simulink model "air_quad"  (R2022b)
settings: Solver=FixedStepDiscrete  StartTime=0.0  StopTime=20  FixedStep=0.01  RelTol=1e-3
model workspace (MAT data in the model file):
  air_quad_config.schema_version = '0.3'
  air_quad_config.plane_model_id = 'quad_sim_b_workbook_b40_v1'
  air_quad_config.power_model_id = 'bench_workbook_fit_v1'
  air_quad_config.power_source = 'bench_synth'
  air_quad_config.mass_kg = 9.581
  air_quad_config.gravity_mps2 = 9.81
  air_quad_config.arm_m = 1
  air_quad_config.rotor_radius_m = 0.508
  air_quad_config.rotor_angle_rad = [0.785398163397; 2.35619449019; 3.92699081699; 5.49778714378]
  air_quad_config.rotor_direction = [1; -1; 1; -1]
  air_quad_config.inertia_kgm2 = [1.3866475  0  0; 0  1.3866475  0; 0  0  2.8184016]
  air_quad_config.pwm_min_us = 1000
  air_quad_config.pwm_max_us = 2000
  air_quad_config.motor_tau_s = 0.08
  air_quad_config.rotor_advance_power_gain = 0
  air_quad_config.rotor_axial_power_gain = 0
  air_quad_config.cm_Nm_per_rad2 = 0.00010188
  air_quad_config.air_density_kgpm3 = 1.225
  air_quad_config.drag_coefficient = [1; 1; 1.1]
  air_quad_config.drag_area_m2 = [0.3; 0.3; 0.273]
  air_quad_config.aux_power_W = 15
  air_quad_config.max_power_W = 2850
  air_quad_config.prop_diameter_m = 1.016
  air_quad_config.h3_induced_gain = 1
  air_quad_config.battery_capacity_Ah = 96
  air_quad_config.battery_n_ser = 7
  air_quad_config.battery_n_par = 4
  air_quad_config.battery_cutoff_V = 16.1
  air_quad_config.battery_r_cell_ohm = 0.012
  air_quad_config.omega_max_radps = 269.443929923
  air_quad_config.pwm_edge_us = 5
  air_quad_config.max_soc = 1
  air_quad_config.min_soc = 0
  air_quad_config.sample_time_s = 0.01
  air_quad_config.speed_rate_mps2 = 2
  air_quad_config.kp_speed = 0.35
  air_quad_config.pitch_max_deg = 25
  air_quad_config.kvz_damp = 0.5
  air_quad_config.kp_att = 25
  air_quad_config.kd_att = 10
  air_quad_config.kp_yaw = 2
  air_quad_config.placeholder = 1
  air_quad_config.placeholder_tag = 'workbook_baseline_20261011'
  air_quad_config.battery_resistance_ohm = 0.021
  air_quad_config.ctrl_period_s = 0
  air_quad_config.cmd_delay_s = 0
  air_quad_config.meas_delay_s = 0
  air_quad_config.meas_noise_V_pct = 0
  air_quad_config.meas_noise_I_pct = 0
  air_quad_config.pwm_slew_us_per_s = 0
  air_quad_config.pwm_quant_us = 0
  air_quad_config.est_delay_s = 0
  air_quad_config.est_noise_pct = 0
  air_quad_config.est_model = 'vi'
  air_quad_config.ctrl_ff_model = 'airspeed'
  air_quad_config.battery_ocv_soc = [0; 0.05; 0.1; 0.15; 0.2; 0.25; 0.3; 0.35; 0.4; 0.45; 0.5; 0.55; 0.6; 0.65; 0.7; 0.75; 0.8; 0.85; 0.9; 0.95; 1]
  air_quad_config.battery_ocv_cell_V = [2.8; 2.88816269848; 2.91644177509; 2.95273554967; 2.99859149086; 3.05539573333; 3.1240653031; 3.20467069632; 3.29608117128; 3.39578047646; 3.5; 3.60421952354; 3.70391882872; 3.79532930368; 3.8759346969; 3.94460426667; 4.00140850914; 4.04726445033; 4.08355822491; 4.11183730152; 4.2]
  air_quad_config.bench_V_nom = 24
  air_quad_config.bench_P_coef = [132.208565 -468.986418 768.635032 -411.475581]
  air_quad_config.bench_T_coef_desc = [0.877076 0 0]
  air_quad_config.ceiling_kn_rpm_per_V = 107.208333333
  air_quad_config.kv_rpm_per_V = 107.208333333
  cmd_reset = [0 0.01 0.02 0.03 0.04 0.05 0.06 0.07 0.08 0.09 0.1 0.11 ... (4002 elements, 2001x2)]
  cmd_vref = [0 0.01 0.02 0.03 0.04 0.05 0.06 0.07 0.08 0.09 0.1 0.11 ... (4002 elements, 2001x2)]
  cmd_wind = [0 0.01 0.02 0.03 0.04 0.05 0.06 0.07 0.08 0.09 0.1 0.11 ... (8004 elements, 2001x4)]
settings Model: Creator=10444  LastModifiedBy=10444

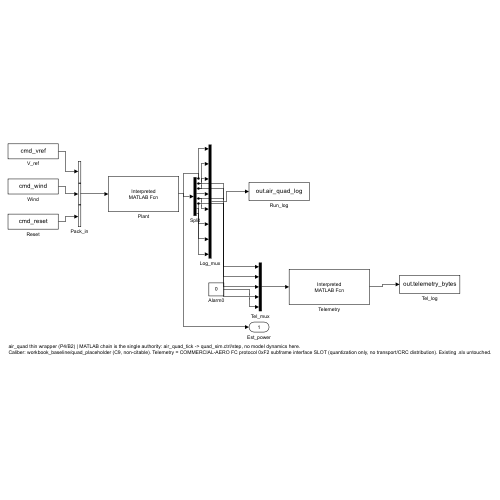
[thumbnail: Simulink's stored preview of the top-level diagram]
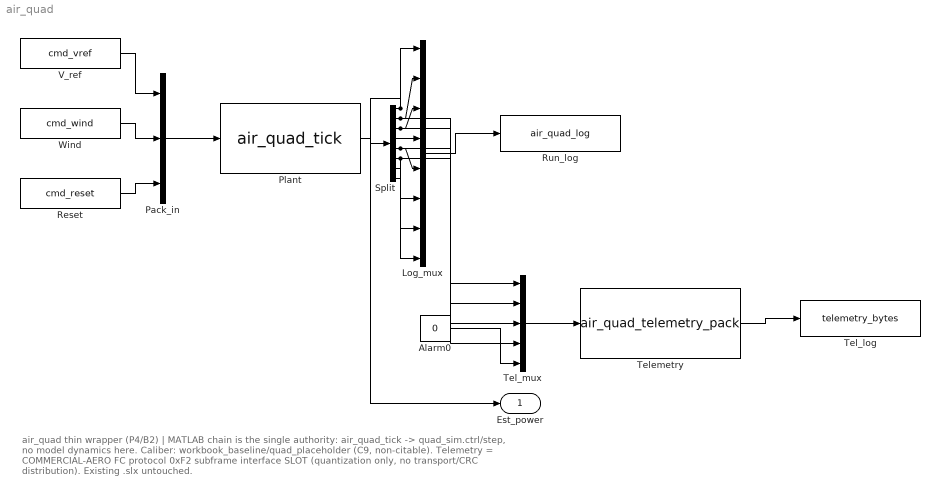
== system air_quad ==
  note: air_quad thin wrapper (P4/B2) | MATLAB chain is the single authority: air_quad_tick -> quad_sim.ctrl/step, no model dynamics here.
      | Caliber: workbook_baseline/quad_placeholder (C9, non-citable). Telemetry = COMMERCIAL-AERO FC protocol 0xF2 subframe interface SLOT (quantization only, no transport/CRC distribution). Existing .slx untouched.
  Alarm0 : Constant  Value=0
  Log_mux : Mux  Inputs=8
  Pack_in : Concatenate  NumInputs=3
  Plant : MATLABFcn  MATLABFcn=air_quad_tick  OutputDimensions=[8]
  Reset : FromWorkspace  VariableName=cmd_reset  Interpolate=off  OutputAfterFinalValue=Holding final value
  Run_log : ToWorkspace  VariableName=air_quad_log  SampleTime=-1
  Split : Demux  Outputs=8
  Tel_log : ToWorkspace  VariableName=telemetry_bytes  SampleTime=-1
  Tel_mux : Mux  Inputs=5
  Telemetry : MATLABFcn  MATLABFcn=air_quad_telemetry_pack  OutputDimensions=[24]
  V_ref : FromWorkspace  VariableName=cmd_vref  Interpolate=off  OutputAfterFinalValue=Holding final value
  Wind : FromWorkspace  VariableName=cmd_wind  Interpolate=off  OutputAfterFinalValue=Holding final value
  Est_power : Outport
  wires:
  V_ref/1 -> Pack_in/1
  Wind/1 -> Pack_in/2
  Reset/1 -> Pack_in/3
  Pack_in/1 -> Plant/1
  Plant/1 -> Split/1
  Split/1 -> Log_mux/1, Est_power/1
  Split/2 -> Log_mux/2, Tel_mux/1
  Split/3 -> Log_mux/3, Tel_mux/2
  Split/4 -> Log_mux/4
  Split/5 -> Log_mux/5, Tel_mux/3
  Split/6 -> Log_mux/6, Tel_mux/4
  Split/7 -> Log_mux/7
  Split/8 -> Log_mux/8
  Log_mux/1 -> Run_log/1
  Alarm0/1 -> Tel_mux/5
  Tel_mux/1 -> Telemetry/1
  Telemetry/1 -> Tel_log/1
